simulink model "LQR_simu"  (R2025a)
settings: Solver=FixedStepAuto  StartTime=0.0  StopTime=4  FixedStep=20e-3  RelTol=1e-3
settings Model: Creator=thepr  LastModifiedBy=thepr

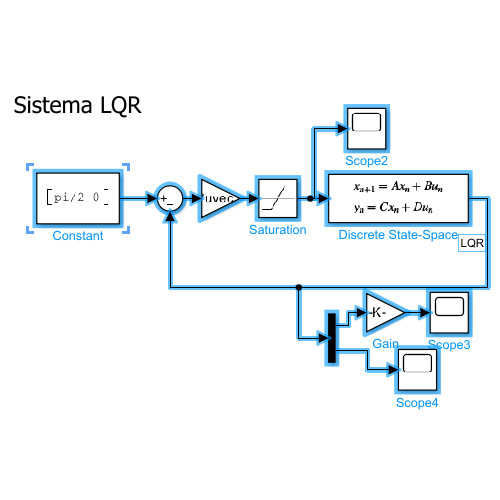
[thumbnail: Simulink's stored preview of the top-level diagram]
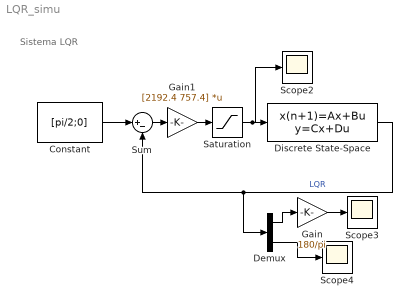
== system LQR_simu ==
  note: Sistema LQR
  Constant : Constant  Value=[pi/2;0]  SampleTime=20e-3
  Demux : Demux  Outputs=2
  Discrete State-Space : DiscreteStateSpace  A=[1 0.0196;0 0.9604]  B=[1e-4*0.0051;1e-4*0.5045]  C=eye(2)  D=[0 ;0]  SampleTime=20e-3
  Gain : Gain  Gain=180/pi
  Gain1 : Gain  Gain=[2192.4 757.4]  Multiplication=Matrix(K*u) (u vector)
  Saturation : Saturate  UpperLimit=4095  LowerLimit=-4095
  Scope2 : Scope
      settings: ActiveDisplayYMinimum=-514.3876517918344  ActiveDisplayYMaximum=3883.614035604794  DataLoggingVariableName=ScopeData2
  Scope3 : Scope
      settings: ActiveDisplayYMinimum=-11.351529689944522  ActiveDisplayYMaximum=102.16376720950072  DataLoggingVariableName=ScopeData3
  Scope4 : Scope
      settings: ActiveDisplayYMinimum=-0.21091417850221092  ActiveDisplayYMaximum=1.7573278410890731  DataLoggingVariableName=ScopeData4
  Sum : Sum  Inputs=|+-
  wires:
  Sum/1 -> Gain1/1
  Discrete State-Space/1 -> Demux/1, Sum/2  "LQR"
  Constant/1 -> Sum/1
  Saturation/1 -> Scope2/1, Discrete State-Space/1
  Gain1/1 -> Saturation/1
  Demux/2 -> Scope4/1
  Gain/1 -> Scope3/1
  Demux/1 -> Gain/1
